simulink model "motor_transfer_function"  (R2025a)
settings: Solver=VariableStepAuto  StartTime=0.0  StopTime=0.4  RelTol=1e-3
undefined symbols (not defined in the file): B_m, denom, J_m, kfi, L_a, num, numI, R_a, T_nl, V_an
settings Model: Creator=kisca  LastModifiedBy=SCH 2

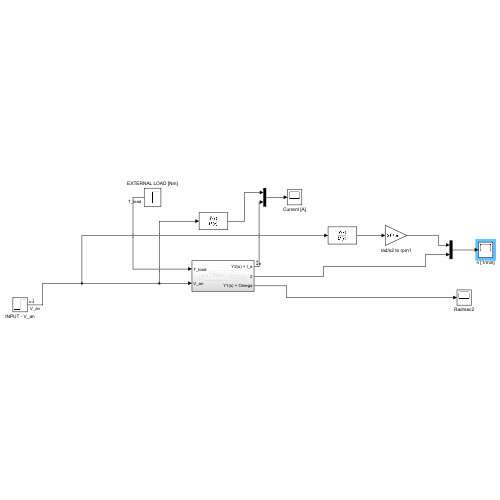
[thumbnail: Simulink's stored preview of the top-level diagram]
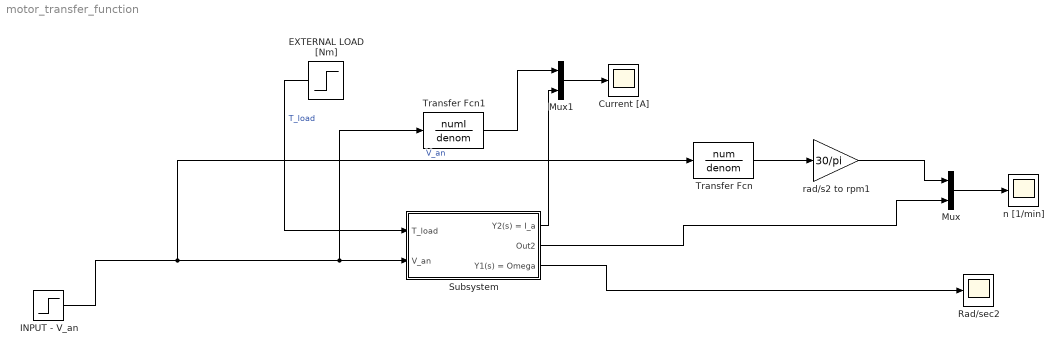
== system motor_transfer_function ==
  Current [A] : Scope
      settings: ActiveDisplayYMinimum=-2.5319338648101777  ActiveDisplayYMaximum=8.8918776629015319
  EXTERNAL LOAD [Nm] : Step  Time=0.25  After=T_nl  SampleTime=0
  INPUT - V_an : Step  Time=0.1  After=V_an  SampleTime=0
  Mux : Mux  Inputs=2
  Mux1 : Mux  Inputs=2
  Rad/sec2 : Scope
      settings: ActiveDisplayYMinimum=-1003.34737  ActiveDisplayYMaximum=9030.12631
  Subsystem : Subsystem
  Transfer Fcn : TransferFcn  Numerator=num  Denominator=denom
  Transfer Fcn1 : TransferFcn  Numerator=numI  Denominator=denom
  n [1/min] : Scope
      settings: ActiveDisplayYMinimum=-944.33038381432652  ActiveDisplayYMaximum=8498.9734543289414  DataLoggingVariableName=ScopeData2
  rad/s2 to rpm1 : Gain  Gain=30/pi
  wires:
  EXTERNAL LOAD [Nm]/1 -> Subsystem/1(T_load)  "T_load"
  INPUT - V_an/1 -> Transfer Fcn/1, Transfer Fcn1/1, Subsystem/2(V_an)  "V_an"
  Subsystem/3(Y1(s) = Omega) -> Rad/sec2/1
  Transfer Fcn/1 -> rad/s2 to rpm1/1
  rad/s2 to rpm1/1 -> Mux/1
  Subsystem/2(Out2) -> Mux/2
  Mux/1 -> n [1/min]/1
  Transfer Fcn1/1 -> Mux1/1
  Subsystem/1(Y2(s) = I_a) -> Mux1/2
  Mux1/1 -> Current [A]/1

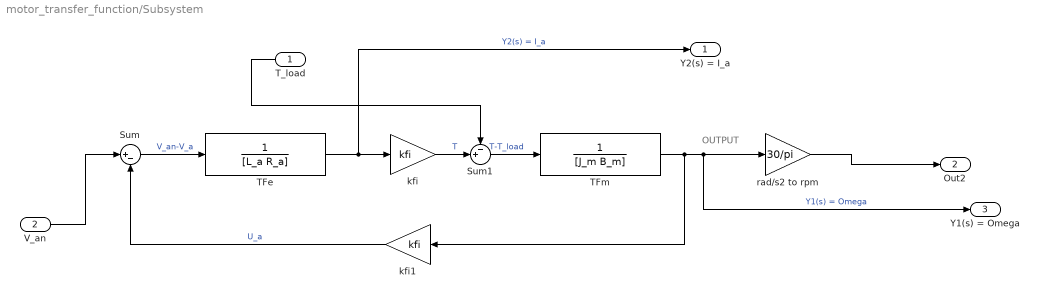
== system motor_transfer_function/Subsystem ==
  note: OUTPUT
  T_load : Inport
  V_an : Inport  Port=2
  Sum : Sum  Inputs=|+-
  Sum1 : Sum  Inputs=-+|
  TFe : TransferFcn  Denominator=[L_a R_a]
  TFm : TransferFcn  Denominator=[J_m B_m]
  kfi : Gain  Gain=kfi
  kfi1 : Gain  Gain=kfi
  rad/s2 to rpm : Gain  Gain=30/pi
  Y2(s) = I_a : Outport
  Out2 : Outport  Port=2
  Y1(s) = Omega : Outport  Port=3
  wires:
  T_load/1 -> Sum1/1
  V_an/1 -> Sum/1
  kfi1/1 -> Sum/2  "U_a"
  TFe/1 -> Y2(s) = I_a/1, kfi/1  "Y2(s) = I_a"
  TFm/1 -> rad/s2 to rpm/1, Y1(s) = Omega/1, kfi1/1  "Y1(s) = Omega"
  kfi/1 -> Sum1/2  "T"
  Sum/1 -> TFe/1  "V_an-V_a"
  Sum1/1 -> TFm/1  "T-T_load"
  rad/s2 to rpm/1 -> Out2/1
